simulink model "IntentOfRUSTRADO_SIH"  (R2026b)
settings: Solver=ode4  StopTime=tf  FixedStep=0.01  EnableMultiTasking=on
undefined symbols (not defined in the file): ArmConstants, DiscIntNeverNeededParam, HexaConstants, st
settings Model: Creator=Carlos Fabian  LastModifiedBy=cfmm
settings SolverCC: PositivePriorityOrder=on
settings OptimizationCC: DifferentSizesBufferReuse=on  EfficientTunableParamExpr=on  EnhancedBackFolding=on  MaxStackSize=64  OptimizationCustomize=off  OptimizeBlockOrder=speed  PassReuseOutputArgsAs=Individual arguments  RemoveInternalMemoryZeroInit=on  RemoveRootLevelIOMemoryZeroInit=on
settings DebuggingCC: ParameterTunabilityLossMsg=error
settings HardwareCC: ProdHWDeviceType=ARM Compatible->ARM Cortex  ProdLargestAtomicFloat=Double  ProdLargestAtomicInteger=Long  ProdLongLongMode=on
settings SFSimCC: MATLABDynamicMemAlloc=off  SimTargetLang=C++
settings RTWCC: Description=Embedded Coder  HardwareBoard=PX4 Host Target  PortableWordSizes=on  SystemTargetFile=ert.tlc  TLCOptions="-aInlineSetEventsForThisBaseRateFcn=TLC_FALSE -aSuppressMultiTaskScheduler=TLC_FALSE  -aRateBasedStepFcn=0"  TargetLang=C++  TemplateMakefile=ert_default_tmf  Toolchain=GNU Tools for PX4 Autopilots
settings CodeAppCC: ForceParamTrailComments=on  IgnoreCustomStorageClasses=off  InsertBlockDesc=on  OperatorAnnotations=on  SFDataObjDesc=on  SimulinkDataObjDesc=on
settings ERTTargetCC: CombineSignalStateStructs=on  ExtModeIntrfLevel=Level2 - Open  ExtModeMexFile=ext_xcp  ExtModeStaticAlloc=on  SupportContinuousTime=on
settings SimscapeCC: SimscapeLogType=all  SimscapeNominalValues="[{\"value\":\"1\",\"unit\":\"A\"},{\"value\":\"1\",\"unit\":\"bar\"},{\"value\":\"1\",\"unit\":\"cm^2\"},{\"value\":\"1\",\"unit\":\"cm^3/s\"},{\"value\":\"1\",\"unit\":\"kJ/kg\"},{\"value\":\"1\",\"unit\":\"kW\"},{\"value\":\"1\",\"unit\":\"l\"},{\"value\":\"1\",\"unit\":\"N\"},{\"value\":\"1\",\"unit\":\"N*m\"},{\"value\":\"1\",\"unit\":\"V\"},{\"value\":\"0.001\",\"unit\":\"Wb\"}]"  SimscapeUseEnergyAccounting=off
settings ExplorerConfigSet: InternalSimMechanicsExplorerSettings=|
  | <ExplorerConfiguration>
  | 
  |   <canonicalview>default</canonicalview>
  | 
  |   <TilePanel>
  |     <TileInfo>
  |       <Tiles Columns="1" Count="1" Height="513" Rows="1" Width="774">
  |         <Row Weight="1"/>
  |         <Column Weight="1"/>
  |         <Tile Height="1" Width="1" X="0" Y="0"/>
  |       </Tiles>
  |     </TileInfo>
  |     <SceneInfo>
  |       <SceneViewer>
  |         <IsThisViewStd>
  |           <IsStandardView>off</IsStandardView>
  |           <StandardViewName>Front</StandardViewName>
  |         </IsThisViewStd>
  |         <BGColor>
  |           <R>1</R>
  |           <G>1</G>
  |           <B>1</B>
  |           <A>1</A>
  |         </BGColor>
  |         <Camera>
  |           <DoPerspective>off</DoPerspective>
  |           <Position>
  |             <X>16.201091586104312</X>
  |             <Y>-16.65504514146788</Y>
  |             <Z>17.087073385082522</Z>
  |           </Position>
  |           <Center>
  |             <X>-0.25720946651222221</X>
  |             <Y>-0.19674408885134653</Y>
  |             <Z>0.62877233246599318</Z>
  |           </Center>
  |           <Up>
  |             <X>-0.40824829046386302</X>
  |             <Y>0.40824829046386302</Y>
  |             <Z>0.81649658092772615</Z>
  |           </Up>
  |           <XLim>2.5491252053936631</XLim>
  |           <YLim>2.5491252053936631</YLim>
  |           <ViewLimDist>0.01</ViewLimDist>
  |         </Camera>
  |       </SceneViewer>
  |     </SceneInfo>
  |   </TilePanel>
  | 
  |   <MechEditorPanel>
  |     <GfxPanelCameraMap/>
  |     <Cameras/>
  |     <VideoCreator>
  |       <IncludeTiles>All</IncludeTiles>
  |       <IncludeTime>on</IncludeTime>
  |       <IncludeWorldFrame>off</IncludeWorldFrame>
  |       <PlaybackSpeedRatio>8</PlaybackSpeedRatio>
  |       <FrameRate>24</FrameRate>
  |       <FrameSize>auto</FrameSize>
  |       <VideoFormat>MotionJPEGAVI</VideoFormat>
  |     </VideoCreator>
  |   </MechEditorPanel>
  | 
  |   <PlaybackSettings>
  |     <PlaybackSpeedFactor>16</PlaybackSpeedFactor>
  |   </PlaybackSettings>
  | 
  | </ExplorerConfiguration>

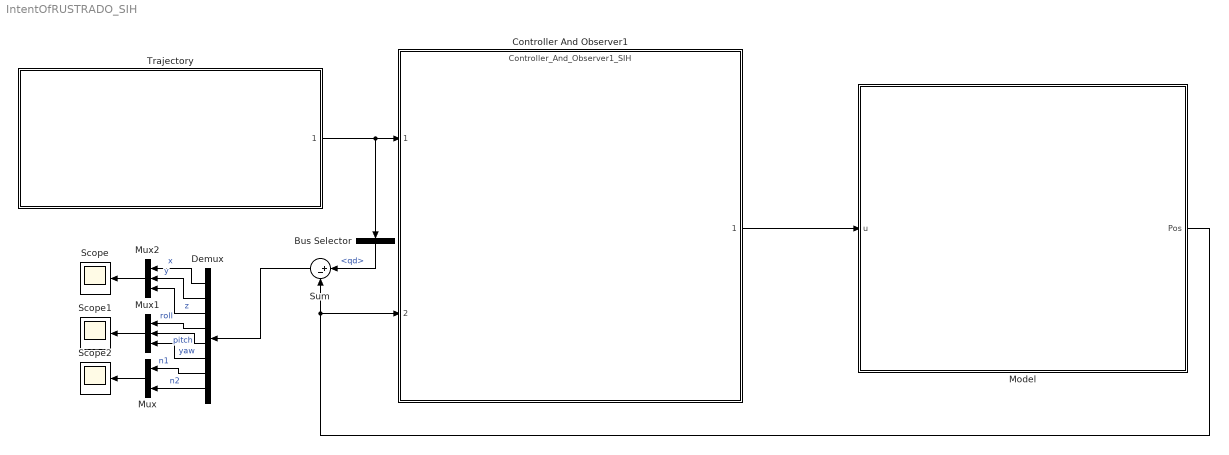
== system IntentOfRUSTRADO_SIH ==
  Bus Selector : BusSelector  OutputSignals=qd
  Controller And Observer1 : ModelReference  ModelNameDialog=Controller_And_Observer1_SIH  SimulationMode=Normal  ModelReferenceVersion=2.6
  Demux : Demux  Outputs=8
  Model : Subsystem
  Mux : Mux  Inputs=2
  Mux1 : Mux  Inputs=3
  Mux2 : Mux  Inputs=3
  Scope : Scope
      settings: ActiveDisplayYMinimum=4.7126799381494294E+117  ActiveDisplayYMaximum=5.6241133109824712E+118
  Scope1 : Scope
      settings: ActiveDisplayYMinimum=-0.00621682249259307  ActiveDisplayYMaximum=0.012057716917689382
  Scope2 : Scope
      settings: ActiveDisplayYMinimum=-0.033824684374711443  ActiveDisplayYMaximum=0.027672278232653655  DataLoggingVariableName=ScopeData2
  Sum : Sum  Inputs=|+-
  Trajectory : Subsystem  ReferencedSubsystem=TrajectoryGeneration
  wires:
  Trajectory/1 -> Controller And Observer1/1, Bus Selector/1
  Model/1(Pos) -> Controller And Observer1/2, Sum/2
  Bus Selector/1 -> Sum/1  "<qd>"
  Sum/1 -> Demux/1
  Mux2/1 -> Scope/1
  Mux1/1 -> Scope1/1
  Mux/1 -> Scope2/1
  Demux/1 -> Mux2/1  "x"
  Demux/2 -> Mux2/2  "y"
  Demux/3 -> Mux2/3  "z"
  Demux/4 -> Mux1/1  "roll"
  Demux/5 -> Mux1/2  "pitch"
  Demux/6 -> Mux1/3  "yaw"
  Demux/7 -> Mux/1  "n1"
  Demux/8 -> Mux/2  "n2"
  Controller And Observer1/1 -> Model/1(u)

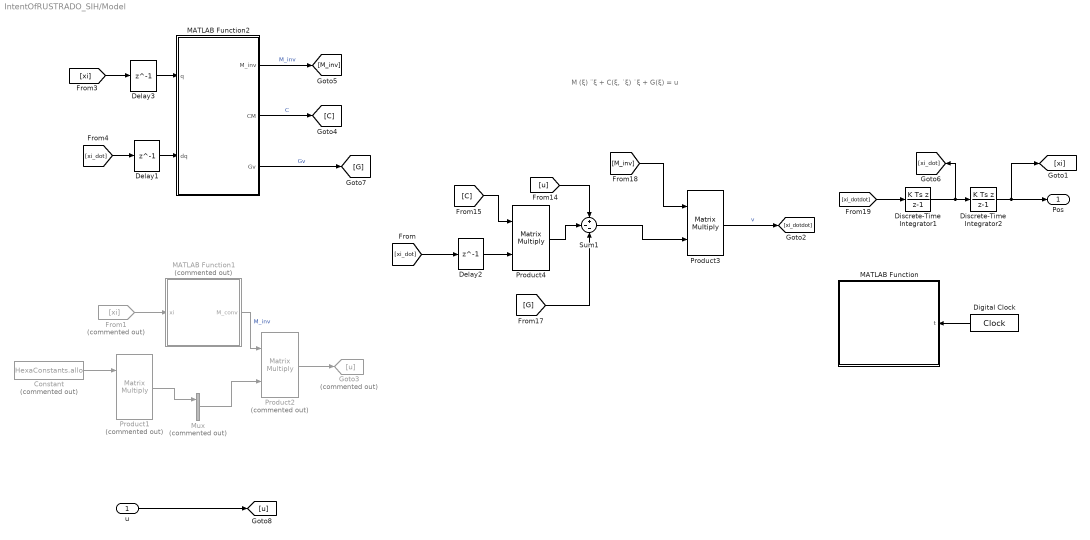
== system IntentOfRUSTRADO_SIH/Model ==
  note: M (ξ) ¨ξ + C(ξ, ˙ξ) ˙ξ + G(ξ) = u
  u : Inport
  Constant : Constant  Commented=on  Value=HexaConstants.allo
  Delay1 : Delay  DelayLength=1  InitialCondition=0  SampleTime=0.01
  Delay2 : Delay  DelayLength=1  InitialCondition=0  SampleTime=0.01
  Delay3 : Delay  DelayLength=1  InitialCondition=0  SampleTime=0.01
  Digital Clock : DigitalClock  SampleTime=0.01
  Discrete-Time Integrator1 : DiscreteIntegrator  IntegratorMethod=Integration: Backward Euler  InitialCondition=zeros(8,1)  SampleTime=st  ICPrevOutput=DiscIntNeverNeededParam  ICPrevScaledInput=DiscIntNeverNeededParam
  Discrete-Time Integrator2 : DiscreteIntegrator  IntegratorMethod=Integration: Backward Euler  InitialCondition=zeros(8,1)  SampleTime=st  ICPrevOutput=DiscIntNeverNeededParam  ICPrevScaledInput=DiscIntNeverNeededParam
  From1 : From  Commented=on  GotoTag=xi
  Goto3 : Goto  Commented=on  GotoTag=u
  MATLAB Function : MATLAB Function  TreatAsAtomicUnit=on
  MATLAB Function1 : MATLAB Function  Commented=on  TreatAsAtomicUnit=on
  MATLAB Function2 : MATLAB Function  TreatAsAtomicUnit=on
  Mux : Mux  Commented=on  Inputs=2
  Product1 : Product  Commented=on  Multiplication=Matrix(*)
  Product2 : Product  Commented=on  Multiplication=Matrix(*)
  Product3 : Product  Multiplication=Matrix(*)
  Product4 : Product  Multiplication=Matrix(*)
  Sum1 : Sum  Inputs=+--
  Pos : Outport  SampleTime=0.01
  wires:
  Discrete-Time Integrator2/1 -> [xi], Pos/1
  [u] -> Sum1/1
  [C] -> Product4/1
  [G] -> Sum1/3
  Sum1/1 -> Product3/2
  [M_inv] -> Product3/1
  Product4/1 -> Sum1/2
  Product3/1 -> [xi_dotdot]  "v"
  [xi_dotdot] -> Discrete-Time Integrator1/1
  Discrete-Time Integrator1/1 -> Discrete-Time Integrator2/1, [xi_dot]
  Digital Clock/1 -> MATLAB Function/1(t)
  MATLAB Function2/3(Gv) -> [G]  "Gv"
  MATLAB Function2/2(CM) -> [C]  "C"
  MATLAB Function2/1(M_inv) -> [M_inv]  "M_inv"
  [xi] -> Delay3/1
  [xi_dot] -> Delay1/1
  [xi_dot] -> Delay2/1
  u/1 -> [u]
  Constant/1 -> Product1/1
  Product1/1 -> Mux/1
  Mux/1 -> Product2/2
  Product2/1 -> Goto3/1
  MATLAB Function1/1(M_conv) -> Product2/1  "M_inv"
  From1/1 -> MATLAB Function1/1(xi)
  Delay3/1 -> MATLAB Function2/1(q)
  Delay1/1 -> MATLAB Function2/2(dq)
  Delay2/1 -> Product4/2

== matlab function IntentOfRUSTRADO_SIH/Model/MATLAB Function2 ==
  data: q input; dq input; HexaConstants parameter; M_inv output; CM output; Gv output; ArmConstants parameter
function [M_inv, CM, Gv] = Get_DCG_Hexa(q, dq, HexaConstants, ArmConstants)

DM = DMatrix(q, HexaConstants, ArmConstants);
CM = CMatrix(q, dq, HexaConstants, ArmConstants);
Gv = GVector(q, HexaConstants, ArmConstants);

M_inv = inv(DM);

end

== matlab function IntentOfRUSTRADO_SIH/Model/MATLAB Function1 ==
  data: xi input; M_conv output
function M_conv  = Get_DCG_Hexa(xi)

phi = xi(4);
theta = xi(5);
psi = xi(6);

C_phi = cos(phi);
S_phi = sin(phi);
    
C_theta = cos(theta);
S_theta = sin(theta);
    
C_psi = cos(psi);
S_psi = sin(psi);

Rb = [
C_psi*C_theta,  C_psi*S_phi*S_theta - C_phi*S_psi,  S_phi*S_psi + C_phi*C_psi*S_theta;
C_theta*S_psi,  C_phi*C_psi + S_psi*S_theta*S_phi, -C_psi*S_phi + S_psi*S_theta*C_phi;
-S_theta,        C_theta*S_phi,                      S_theta*C_phi
];

W = [
1,       0,        -S_theta;
0,   C_phi,  C_theta*S_phi;
0,  -S_phi,  C_theta*C_phi
];

w_inv = inv(W);

M_conv = [Rb, zeros(3,3), zeros(3,2);
    zeros(3,3), w_inv, zeros(3,2);
    zeros(2,3), zeros(2,3), eye(2)];

end

== matlab function IntentOfRUSTRADO_SIH/Model/MATLAB Function ==
  data: t input; PickObj parameter
function GetPickObj(t, PickObj)

Times = PickObj.Time;

if length(Times) == 2
    cond = t <= Times(1) || t >= Times(2);
else
    cond = t <= Times(1);
end

if ~cond
    m = PickObj.Mass;
    r = PickObj.Radius;
    I1 = 2/5*m*r^2;
    I = diag([I1, I1, I1]);
else
    m = 0;
    I = zeros(3, 3);
end

end
